simulink model "PMSMHighFrequencyPlant"  (R2026b)
settings: Solver=VariableStepAuto
undefined symbols (not defined in the file or in its folder): hfPlantCfg
settings Model: Creator=24322  LastModifiedBy=24322

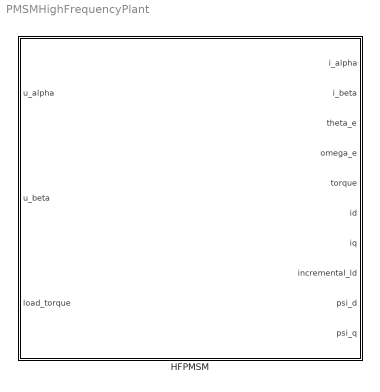
== system PMSMHighFrequencyPlant ==
  HFPMSM : Subsystem  mask{cfg=hfPlantCfg}
      mask prompts: cfg "PMSM physical configuration"

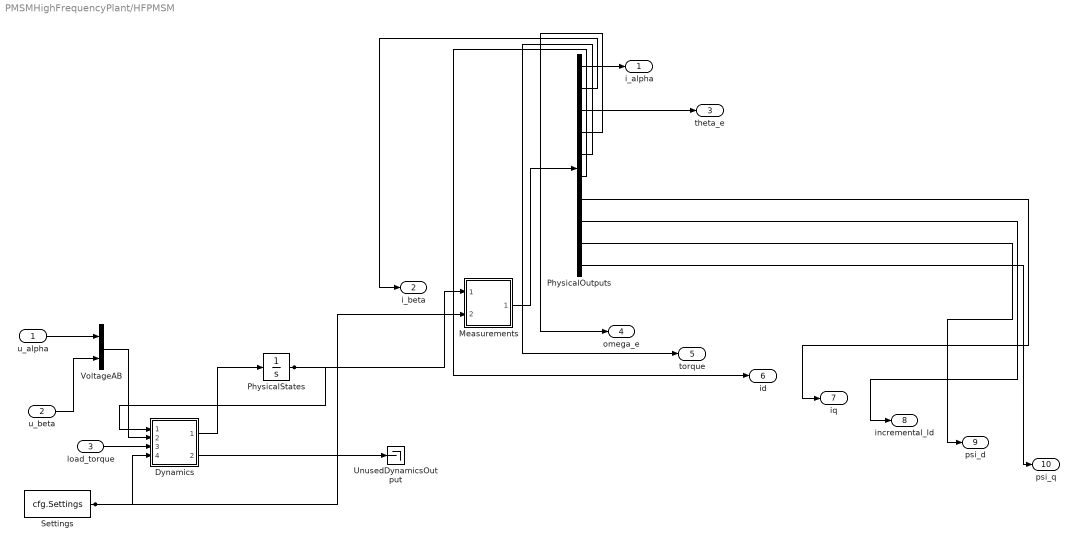
== system PMSMHighFrequencyPlant/HFPMSM ==
  u_alpha : Inport
  u_beta : Inport  Port=2
  load_torque : Inport  Port=3
  Dynamics : MATLAB Function  TreatAsAtomicUnit=on
  Measurements : MATLAB Function  TreatAsAtomicUnit=on
  PhysicalOutputs : Demux  Outputs=10
  PhysicalStates : Integrator  InitialCondition=cfg.InitialState
  Settings : Constant  Value=cfg.Settings
  UnusedDynamicsOutput : Terminator
  VoltageAB : Mux  Inputs=2
  i_alpha : Outport
  i_beta : Outport  Port=2
  theta_e : Outport  Port=3
  omega_e : Outport  Port=4
  torque : Outport  Port=5
  id : Outport  Port=6
  iq : Outport  Port=7
  incremental_ld : Outport  Port=8
  psi_d : Outport  Port=9
  psi_q : Outport  Port=10
  wires:
  u_beta/1 -> VoltageAB/2
  u_alpha/1 -> VoltageAB/1
  Measurements/1(signals) -> PhysicalOutputs/1
  PhysicalStates/1 -> Dynamics/1(state), Measurements/1(state)
  VoltageAB/1 -> Dynamics/2(voltage)
  load_torque/1 -> Dynamics/3(loadTorque)
  Settings/1 -> Measurements/2(settings), Dynamics/4(settings)
  Dynamics/1(derivative) -> PhysicalStates/1
  Dynamics/2(signals) -> UnusedDynamicsOutput/1
  PhysicalOutputs/1 -> i_alpha/1
  PhysicalOutputs/2 -> i_beta/1
  PhysicalOutputs/3 -> theta_e/1
  PhysicalOutputs/4 -> omega_e/1
  PhysicalOutputs/5 -> torque/1
  PhysicalOutputs/6 -> id/1
  PhysicalOutputs/7 -> iq/1
  PhysicalOutputs/8 -> incremental_ld/1
  PhysicalOutputs/9 -> psi_d/1
  PhysicalOutputs/10 -> psi_q/1

== matlab function PMSMHighFrequencyPlant/HFPMSM/Measurements ==
  data: state input; signals output; settings input
function signals=pmsm_hf_output(state,settings)
%PMSM_HF_OUTPUT State-only sensor outputs, with no applied-voltage feedthrough.
% Reuse the identical magnetic equations; discard the dummy-voltage derivative.
%#codegen
[~,signals]=pmsm_hf_dynamics(state,zeros(2,1,'like',state),zeros(1,'like',state),settings);
end

== matlab function PMSMHighFrequencyPlant/HFPMSM/Dynamics ==
  data: state input; derivative output; voltage input; loadTorque input; settings input; signals output
function [derivative,signals]=pmsm_hf_dynamics(state,voltage,loadTorque,settings)
%PMSM_HF_DYNAMICS Continuous nonlinear salient PMSM in physical rotor dq axes.
% state=[id;iq;omega_mechanical;theta_mechanical], voltage=[u_alpha;u_beta].
% settings=[Rs;Ld0;Lq;Flux;p;J;B;SaturationDepth;SaturationCurrent;M;MechanicalEnabled].
% psi_d=Flux+Ld0*(id-s*Is*log(cosh(id/Is)))+M*iq, psi_q=Lq*iq+M*id.
% The symmetric differential-inductance matrix is the flux Jacobian.
%#codegen
id=state(1);iq=state(2);speed=state(3);theta=settings(5)*state(4);
x=id/settings(9);absolute=abs(x);
logCosh=absolute+log1p(exp(-2*absolute))-log(2);
psiD=settings(4)+settings(2)*(id-settings(8)*settings(9)*logCosh)+settings(10)*iq;
psiQ=settings(3)*iq+settings(10)*id;
ld=settings(2)*(1-settings(8)*tanh(x));lq=settings(3);mutual=settings(10);
cosine=cos(theta);sine=sin(theta);omega=settings(5)*speed;
vd=cosine*voltage(1)+sine*voltage(2);
vq=-sine*voltage(1)+cosine*voltage(2);
balanceD=vd-settings(1)*id+omega*psiQ;
balanceQ=vq-settings(1)*iq-omega*psiD;
determinant=ld*lq-mutual*mutual;
derivative=zeros(4,1,'like',state);
derivative(1)=(lq*balanceD-mutual*balanceQ)/determinant;
derivative(2)=(ld*balanceQ-mutual*balanceD)/determinant;
torque=1.5*settings(5)*(psiD*iq-psiQ*id);
if settings(11)>0.5
    derivative(3)=(torque-loadTorque-settings(7)*speed)/settings(6);
    derivative(4)=speed;
end
signals=[cosine*id-sine*iq;sine*id+cosine*iq;atan2(sine,cosine);omega; ...
    torque;id;iq;ld;psiD;psiQ];
end
